simulink model "sf_aircontrol_with_atomic_subcharts"  (R2025b)
settings: Solver=ode45  StartTime=0.0  StopTime=600  FixedStep=1000  RelTol=1e-3  EnableMultiTasking=on
libraries: SignalEditorBlockLib x1
settings Model: ExtModeAutoUpdateStatusClock=off  Creator=The MathWorks, Inc.  LastModifiedBy=The MathWorks, Inc.
settings SolverCC: MaxConsecutiveZCs=500  AlgebraicLoopSolver=TrustRegion
settings DataIOCC: LimitDataPoints=on  SaveFormat=Array  ReturnWorkspaceOutputs=off
settings OptimizationCC: ReuseModelBlockBuffer=off  ExpressionDepthLimit=2147483647.0  InitFltsAndDblsToZero=on  LifeSpan=inf
settings DebuggingCC: SaveWithParameterizedLinksMsg=none  UnderspecifiedInitializationDetection=Classic  MergeDetectMultiDrivingBlocksExec=none  SignalResolutionControl=TryResolveAllWithWarning  MultiTaskDSMMsg=warning  MultiTaskCondExecSysMsg=none  FcnCallInpInsideContextMsg=warning  UnconnectedInputMsg=warning  UnconnectedOutputMsg=warning  UnconnectedLineMsg=warning  StateNameClashWarn=warning  SFUnexpectedBacktrackingDiag=warning  SFNoUnconditionalDefaultTransitionDiag=warning  SFExecutionAtInitializationDiag=none  ArithmeticOperatorsInVariantConditions=warning
settings HardwareCC: ProdBitPerPointer=32.0  ProdBitPerSizeT=32.0  ProdBitPerPtrDiffT=32.0  ProdLargestAtomicFloat=None  ProdIntDivRoundTo=Undefined  ProdEndianess=Unspecified  ProdWordSize=32.0  ProdHWDeviceType=32-bit Generic
settings ModelReferenceCC: EnableRefExpFcnMdlSchedulingChecks=on  PropagateSignalLabelsOutOfModel=off
settings SFSimCC: SimUseLocalCustomCode=off  SimParseCustomCode=off
settings RTWCC: RTWUseLocalCustomCode=off  GPUComputeCapability=3.5
settings CodeAppCC: StateflowObjectComments=on
settings GRTTargetCC: TargetFcnLib=ansi_tfl_tmw.mat  TargetLangStandard=C89/C90 (ANSI)  CombineOutputUpdateFcns=off  GRTInterface=on
settings ConfigComp: CovMetricSettings=dw  CovSaveCumulativeToWorkspaceVar=on  CovSaveSingleToWorkspaceVar=on  CovExternalEMLEnable=off

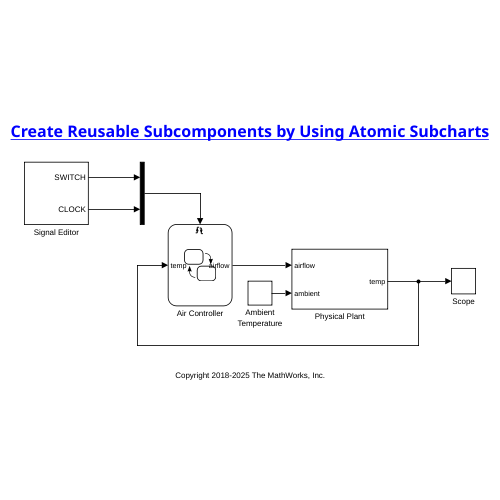
[thumbnail: Simulink's stored preview of the top-level diagram]
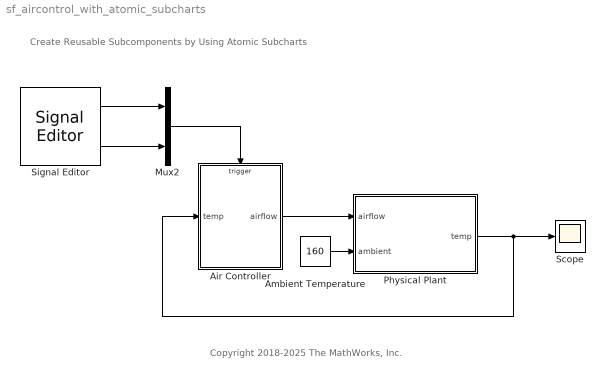
== system sf_aircontrol_with_atomic_subcharts ==
  note: Copyright 2018-2025 The MathWorks, Inc.
  note: Create Reusable Subcomponents by Using Atomic Subcharts
  Air Controller : Stateflow chart  TreatAsAtomicUnit=on
  Ambient Temperature : Constant  Value=160
  Mux2 : Mux  Inputs=2
  Physical Plant : Subsystem
  Scope : Scope
      settings: TimeSpan=600  ActiveDisplayYMinimum=60  ActiveDisplayYMaximum=160
  Signal Editor : SignalEditorBlockLib/Signal Editor  FileName=AirControlInput.mat  ActiveScenario=Group_1  ActiveSignal=CLOCK  IsBus=off  OutputBusObjectStr=Bus: BusObject  SampleTime=0  OutputAfterFinalValue=Extrapolation  Unit=inherit  PreserveSignalName=on  ApplySigPropsToAllScenarios=on  ApplySigPropsToAllSignals=off  SignalPropertySource=Dialog parameters
  wires:
  Mux2/1 -> Air Controller/Trigger
  Air Controller/1(airflow) -> Physical Plant/1(airflow)
  Ambient Temperature/1 -> Physical Plant/2(ambient)
  Physical Plant/1(temp) -> Scope/1, Air Controller/1(temp)
  Signal Editor/1 -> Mux2/1
  Signal Editor/2 -> Mux2/2

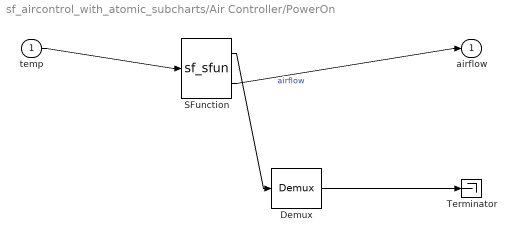
== system sf_aircontrol_with_atomic_subcharts/Air Controller/PowerOn ==
  temp : Inport
  " Demux " : Demux  Outputs=1
  " SFunction " : S-Function  Tag=Stateflow S-Function 3  FunctionName=sf_sfun  PortCounts=[1 2]  SFunctionDeploymentMode=off  EnableBusSupport=off
  " Terminator " : Terminator
  airflow : Outport  VectorParamsAs1DForOutWhenUnconnected=off
  wires:
  temp/1 -> " SFunction "/1
  " SFunction "/2 -> airflow/1  "airflow"
  " Demux "/1 -> " Terminator "/1
  " SFunction "/1 -> " Demux "/1

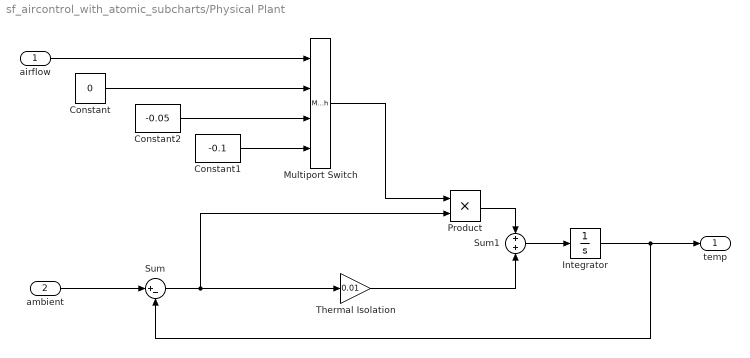
== system sf_aircontrol_with_atomic_subcharts/Physical Plant ==
  airflow : Inport
  ambient : Inport  Port=2
  Constant : Constant  Value=0
  Constant1 : Constant  Value=-0.1
  Constant2 : Constant  Value=-0.05
  Integrator : Integrator  InitialCondition=70
  Multiport Switch : MultiPortSwitch  DataPortOrder=Zero-based contiguous  zeroidx=on  SaturateOnIntegerOverflow=off  InputSameDT=off
  Product : Product  RndMeth=Zero
  Sum : Sum  Inputs=|+-
  Sum1 : Sum  Inputs=+|+
  Thermal Isolation : Gain  Gain=0.01
  temp : Outport  VectorParamsAs1DForOutWhenUnconnected=off
  wires:
  Integrator/1 -> temp/1, Sum/2
  Sum1/1 -> Integrator/1
  Constant2/1 -> Multiport Switch/3
  Constant/1 -> Multiport Switch/2
  airflow/1 -> Multiport Switch/1
  ambient/1 -> Sum/1
  Sum/1 -> Thermal Isolation/1, Product/2
  Product/1 -> Sum1/1
  Thermal Isolation/1 -> Sum1/2
  Multiport Switch/1 -> Product/1
  Constant1/1 -> Multiport Switch/4

== stateflow chart sf_aircontrol_with_atomic_subcharts/Air Controller ==
  state PowerOff
    en:
    airflow = 0;
  state PowerOn
  (default) -> PowerOff
  PowerOn -> PowerOff : SWITCH
  PowerOff -> PowerOn : SWITCH
  data: airflow output uint8; temp input
  events: SWITCH input EITHER_EDGE_EVENT; CLOCK input EITHER_EDGE_EVENT

== stateflow chart sf_aircontrol_with_atomic_subcharts/Air Controller/PowerOn ==
  state FAN1 [parallel]
    settings: executionOrder=1
    state On
    state Off
    FAN1.On -> FAN1.Off : [temp < 120]
    (default) -> FAN1.Off
    FAN1.Off -> FAN1.On : [temp >=120]
  state FAN2 [parallel]
    settings: executionOrder=2
    state On
    state Off
    FAN2.On -> FAN2.Off : [temp<150]
    (default) -> FAN2.Off
    FAN2.Off -> FAN2.On : [temp>=150]
  state SpeedValue [parallel]
    du: airflow = in(FAN1.On) + in(FAN2.On);
    settings: executionOrder=3
  data: airflow output uint8; temp input
